simulink model "rfsoc4x2_ospfb_128"  (R2021a)
settings: Solver=VariableStepAuto  StartTime=0.0  StopTime=2048  RelTol=1e-3
undefined symbols (not defined in the file): pfb_coeff_gen_calc
libraries: xbsIndex_r4 x37092, casper_library_delays x737, casper_library_misc x68, xps_library x1
(part 335 of 339)

== system rfsoc4x2_ospfb_128/fft2/fft_biplex/biplex_core/fft_stage_4/butterfly_direct/twiddle/bus_mult/mult4/a_replicate ==
  in : Inport
  bussify : Subsystem  AncestorBlock=casper_library_flow_control/bus_create  mask(bus_create){inputNum=2}
      mask prompts: inputNum "Number of inputs:"
      mask init:
      | bus_create_init(gcb,...
      |     'inputNum', inputNum);
  out : Outport
  wires:
  bussify/1(bus_out) -> out/1
  in/1 -> bussify/2(in2), bussify/1(in1)

== system rfsoc4x2_ospfb_128/fft2/fft_biplex/biplex_core/fft_stage_4/butterfly_direct/twiddle/bus_mult/mult4/b_expand ==
  bus_in : Inport
  reinterpret{1..4} (4 alike) : xbsIndex_r4/Reinterpret  force_arith_type=on  arith_type="Signed  (2's comp)"  force_bin_pt=on  bin_pt=17  block_type=reinterpret
  slice1 : xbsIndex_r4/Slice  nbits=18  boolean_output=off  mode=Upper Bit Location + Width  bit1=-54  base1=MSB of Input  bit0=0  base0=LSB of Input  dbl_ovrd=off  block_type=slice
  slice2 : xbsIndex_r4/Slice  nbits=18  boolean_output=off  mode=Upper Bit Location + Width  bit1=-36  base1=MSB of Input  bit0=0  base0=LSB of Input  dbl_ovrd=off  block_type=slice
  slice3 : xbsIndex_r4/Slice  nbits=18  boolean_output=off  mode=Upper Bit Location + Width  bit1=-18  base1=MSB of Input  bit0=0  base0=LSB of Input  dbl_ovrd=off  block_type=slice
  slice4 : xbsIndex_r4/Slice  nbits=18  boolean_output=off  mode=Upper Bit Location + Width  bit1=0  base1=MSB of Input  bit0=0  base0=LSB of Input  dbl_ovrd=off  block_type=slice
  msb_out4 : Outport
  out3 : Outport  Port=2
  out2 : Outport  Port=3
  lsb_out1 : Outport  Port=4  VectorParamsAs1DForOutWhenUnconnected=off
  wires:
  reinterpret1/1 -> lsb_out1/1
  slice1/1 -> reinterpret1/1
  reinterpret2/1 -> out2/1
  slice2/1 -> reinterpret2/1
  reinterpret3/1 -> out3/1
  slice3/1 -> reinterpret3/1
  reinterpret4/1 -> msb_out4/1
  slice4/1 -> reinterpret4/1
  bus_in/1 -> slice1/1, slice2/1, slice3/1, slice4/1

== system rfsoc4x2_ospfb_128/fft2/fft_biplex/biplex_core/fft_stage_4/butterfly_direct/twiddle/bus_mult/mult4/b_replicate ==
  in : Inport
  bussify : Subsystem  AncestorBlock=casper_library_flow_control/bus_create  mask(bus_create){inputNum=2}
      mask prompts: inputNum "Number of inputs:"
      mask init:
      | bus_create_init(gcb,...
      |     'inputNum', inputNum);
  out : Outport
  wires:
  bussify/1(bus_out) -> out/1
  in/1 -> bussify/2(in2), bussify/1(in1)

== system rfsoc4x2_ospfb_128/fft2/fft_biplex/biplex_core/fft_stage_4/butterfly_direct/twiddle/bus_mult/mult4/ri_to_c ==
  re : Inport
  im : Inport  Port=2
  concat : xbsIndex_r4/Concat  num_inputs=2  dbl_ovrd=off  block_type=concat
      settings: block_version=9.1.01
  force_im : xbsIndex_r4/Reinterpret  force_arith_type=on  arith_type=Unsigned  force_bin_pt=on  bin_pt=0  block_type=reinterpret
      settings: infoedit="Changes signal type without altering the binary representation.   You can changed the signal between signed and unsigned, and relocate the binary point.<P><P>Hardware notes: In hardware this block costs nothing.<P><P>Example:  Suppose the input is 6 bits wide, signed, with 2 fractional bits, and the output is forced to unsigned with 0 fractional bits.  Then an input of -2.0 (1110.00 in binary 2's complement) becomes an output of 56 (111000 in binary)."  block_version=9.1.01
  force_re : xbsIndex_r4/Reinterpret  force_arith_type=on  arith_type=Unsigned  force_bin_pt=on  bin_pt=0  block_type=reinterpret
      settings: infoedit="Changes signal type without altering the binary representation.   You can changed the signal between signed and unsigned, and relocate the binary point.<P><P>Hardware notes: In hardware this block costs nothing.<P><P>Example:  Suppose the input is 6 bits wide, signed, with 2 fractional bits, and the output is forced to unsigned with 0 fractional bits.  Then an input of -2.0 (1110.00 in binary 2's complement) becomes an output of 56 (111000 in binary)."  block_version=9.1.01
  c : Outport  VectorParamsAs1DForOutWhenUnconnected=off
  wires:
  im/1 -> force_im/1
  concat/1 -> c/1
  re/1 -> force_re/1
  force_im/1 -> concat/2
  force_re/1 -> concat/1

== system rfsoc4x2_ospfb_128/fft2/fft_biplex/biplex_core/fft_stage_4/butterfly_direct/twiddle/bus_mult/repa/bussify ==
  in1 : Inport
  reinterpret1 : xbsIndex_r4/Reinterpret  force_arith_type=on  arith_type=Unsigned  force_bin_pt=on  bin_pt=0  block_type=reinterpret
      settings: infoedit="Changes signal type without altering the binary representation.   You can changed the signal between signed and unsigned, and relocate the binary point.<br><br>Hardware notes: In hardware this block costs nothing.<br><br>Example:  Suppose the input is 6 bits wide, signed, with 2 fractional bits, and the output is forced to unsigned with 0 fractional bits.  Then an input of -2.0 (1110.00 in binary 2's complement) becomes an output of 56 (111000 in binary)."
  bus_out : Outport  VectorParamsAs1DForOutWhenUnconnected=off
  wires:
  reinterpret1/1 -> bus_out/1
  in1/1 -> reinterpret1/1

== system rfsoc4x2_ospfb_128/fft2/fft_biplex/biplex_core/fft_stage_4/butterfly_direct/twiddle/bus_mult/repb/bussify ==
  in1 : Inport
  reinterpret1 : xbsIndex_r4/Reinterpret  force_arith_type=on  arith_type=Unsigned  force_bin_pt=on  bin_pt=0  block_type=reinterpret
      settings: infoedit="Changes signal type without altering the binary representation.   You can changed the signal between signed and unsigned, and relocate the binary point.<br><br>Hardware notes: In hardware this block costs nothing.<br><br>Example:  Suppose the input is 6 bits wide, signed, with 2 fractional bits, and the output is forced to unsigned with 0 fractional bits.  Then an input of -2.0 (1110.00 in binary 2's complement) becomes an output of 56 (111000 in binary)."
  bus_out : Outport  VectorParamsAs1DForOutWhenUnconnected=off
  wires:
  reinterpret1/1 -> bus_out/1
  in1/1 -> reinterpret1/1

== system rfsoc4x2_ospfb_128/fft2/fft_biplex/biplex_core/fft_stage_4/butterfly_direct/twiddle/coeff_gen/cosin/add_convert0 ==
  theta : Inport
  misci : Inport  Port=2
  AddSub5 : xbsIndex_r4/AddSub  mode=Addition  use_carryin=off  use_carryout=off  en=off  latency=0  precision=User Defined  arith_type=Unsigned  n_bits=2  bin_pt=0  quantization=Truncate  overflow=Wrap  use_behavioral_HDL=off  hw_selection=Fabric  pipelined=off  dbl_ovrd=off  block_type=addsub
  Concat : xbsIndex_r4/Concat  num_inputs=2  dbl_ovrd=off  block_type=concat
  Convert2 : xbsIndex_r4/Convert  gui_display_data_type=Fixed-point  arith_type=Unsigned  n_bits=3  bin_pt=0  float_type=Single  exp_bits=8  fraction_bits=24  quantization=Truncate  overflow=Saturate  en=off  latency=conv_latency  pipeline=on  dbl_ovrd=off  block_type=convert
  Delay1 : xbsIndex_r4/Delay  rst=off  infoeditControl=Selection of Reset will increase slice count due to use of real FFs and instead of SRLs  en=off  latency=mux_latency+add_latency+conv_latency  reg_retiming=on  dbl_ovrd=off  block_type=delay
  Delay13 : xbsIndex_r4/Delay  rst=off  infoeditControl=Selection of Reset will increase slice count due to use of real FFs and instead of SRLs  en=off  latency=mux_latency  reg_retiming=on  dbl_ovrd=off  block_type=delay
  Delay14 : xbsIndex_r4/Delay  rst=off  infoeditControl=Selection of Reset will increase slice count due to use of real FFs and instead of SRLs  en=off  latency=add_latency  reg_retiming=off  dbl_ovrd=off  block_type=delay
  Delay2 : xbsIndex_r4/Delay  rst=off  infoeditControl=Selection of Reset will increase slice count due to use of real FFs and instead of SRLs  en=off  latency=add_latency+mux_latency+conv_latency  reg_retiming=on  dbl_ovrd=off  block_type=delay
  direction_offset : xbsIndex_r4/Constant  const=0  gui_display_data_type=Fixed-point  arith_type=Unsigned  n_bits=2  bin_pt=0  preci_type=Single  exp_width=8  frac_width=24  explicit_period=off  period=1  equ=P=C  opselect=C  inp2=PCIN>>17  opr=+  inp1=P  carry=CIN  dbl_ovrd=off  block_type=constant
  fluff : xbsIndex_r4/Concat  num_inputs=2  dbl_ovrd=off  block_type=concat
  invert : xbsIndex_r4/Slice  nbits=1  boolean_output=on  mode=Upper Bit Location + Width  bit1=0  base1=MSB of Input  bit0=0  base0=LSB of Input  dbl_ovrd=off  block_type=slice
  lookup : xbsIndex_r4/Slice  nbits=2  boolean_output=off  mode=Lower Bit Location + Width  bit1=0  base1=MSB of Input  bit0=0  base0=LSB of Input  dbl_ovrd=off  block_type=slice
  new_add : xbsIndex_r4/Slice  nbits=3  boolean_output=off  mode=Lower Bit Location + Width  bit1=0  base1=MSB of Input  bit0=0  base0=LSB of Input  dbl_ovrd=off  block_type=slice
  pad : xbsIndex_r4/Constant  const=0  gui_display_data_type=Fixed-point  arith_type=Unsigned  n_bits=1  bin_pt=0  preci_type=Single  exp_width=8  frac_width=24  explicit_period=off  period=1  equ=P=C  opselect=C  inp2=PCIN>>17  opr=+  inp1=P  carry=CIN  dbl_ovrd=off  block_type=constant
  quadrant : xbsIndex_r4/Slice  nbits=2  boolean_output=off  mode=Upper Bit Location + Width  bit1=0  base1=MSB of Input  bit0=0  base0=LSB of Input  dbl_ovrd=off  block_type=slice
  negate : Outport
  add : Outport  Port=2
  misco : Outport  Port=3
  wires:
  theta/1 -> fluff/2
  pad/1 -> fluff/1
  fluff/1 -> quadrant/1, lookup/1
  direction_offset/1 -> AddSub5/1
  quadrant/1 -> AddSub5/2
  lookup/1 -> Concat/2
  AddSub5/1 -> Concat/1, invert/1
  Concat/1 -> new_add/1
  new_add/1 -> Delay14/1
  Convert2/1 -> add/1
  Delay14/1 -> Delay13/1
  Delay13/1 -> Convert2/1
  invert/1 -> Delay2/1
  Delay2/1 -> negate/1
  misci/1 -> Delay1/1
  Delay1/1 -> misco/1

== system rfsoc4x2_ospfb_128/fft2/fft_biplex/biplex_core/fft_stage_4/butterfly_direct/twiddle/coeff_gen/cosin/add_convert1 ==
  theta : Inport
  misci : Inport  Port=2
  AddSub5 : xbsIndex_r4/AddSub  mode=Addition  use_carryin=off  use_carryout=off  en=off  latency=0  precision=User Defined  arith_type=Unsigned  n_bits=2  bin_pt=0  quantization=Truncate  overflow=Wrap  use_behavioral_HDL=off  hw_selection=Fabric  pipelined=off  dbl_ovrd=off  block_type=addsub
  Concat : xbsIndex_r4/Concat  num_inputs=2  dbl_ovrd=off  block_type=concat
  Convert2 : xbsIndex_r4/Convert  gui_display_data_type=Fixed-point  arith_type=Unsigned  n_bits=3  bin_pt=0  float_type=Single  exp_bits=8  fraction_bits=24  quantization=Truncate  overflow=Saturate  en=off  latency=conv_latency  pipeline=on  dbl_ovrd=off  block_type=convert
  Delay1 : xbsIndex_r4/Delay  rst=off  infoeditControl=Selection of Reset will increase slice count due to use of real FFs and instead of SRLs  en=off  latency=mux_latency+add_latency+conv_latency  reg_retiming=on  dbl_ovrd=off  block_type=delay
  Delay13 : xbsIndex_r4/Delay  rst=off  infoeditControl=Selection of Reset will increase slice count due to use of real FFs and instead of SRLs  en=off  latency=mux_latency  reg_retiming=on  dbl_ovrd=off  block_type=delay
  Delay14 : xbsIndex_r4/Delay  rst=off  infoeditControl=Selection of Reset will increase slice count due to use of real FFs and instead of SRLs  en=off  latency=add_latency  reg_retiming=off  dbl_ovrd=off  block_type=delay
  Delay2 : xbsIndex_r4/Delay  rst=off  infoeditControl=Selection of Reset will increase slice count due to use of real FFs and instead of SRLs  en=off  latency=add_latency+mux_latency+conv_latency  reg_retiming=on  dbl_ovrd=off  block_type=delay
  direction_offset : xbsIndex_r4/Constant  const=0  gui_display_data_type=Fixed-point  arith_type=Unsigned  n_bits=2  bin_pt=0  preci_type=Single  exp_width=8  frac_width=24  explicit_period=off  period=1  equ=P=C  opselect=C  inp2=PCIN>>17  opr=+  inp1=P  carry=CIN  dbl_ovrd=off  block_type=constant
  fluff : xbsIndex_r4/Concat  num_inputs=2  dbl_ovrd=off  block_type=concat
  invert : xbsIndex_r4/Slice  nbits=1  boolean_output=on  mode=Upper Bit Location + Width  bit1=0  base1=MSB of Input  bit0=0  base0=LSB of Input  dbl_ovrd=off  block_type=slice
  lookup : xbsIndex_r4/Slice  nbits=2  boolean_output=off  mode=Lower Bit Location + Width  bit1=0  base1=MSB of Input  bit0=0  base0=LSB of Input  dbl_ovrd=off  block_type=slice
  new_add : xbsIndex_r4/Slice  nbits=3  boolean_output=off  mode=Lower Bit Location + Width  bit1=0  base1=MSB of Input  bit0=0  base0=LSB of Input  dbl_ovrd=off  block_type=slice
  pad : xbsIndex_r4/Constant  const=0  gui_display_data_type=Fixed-point  arith_type=Unsigned  n_bits=1  bin_pt=0  preci_type=Single  exp_width=8  frac_width=24  explicit_period=off  period=1  equ=P=C  opselect=C  inp2=PCIN>>17  opr=+  inp1=P  carry=CIN  dbl_ovrd=off  block_type=constant
  quadrant : xbsIndex_r4/Slice  nbits=2  boolean_output=off  mode=Upper Bit Location + Width  bit1=0  base1=MSB of Input  bit0=0  base0=LSB of Input  dbl_ovrd=off  block_type=slice
  negate : Outport
  add : Outport  Port=2
  misco : Outport  Port=3
  wires:
  theta/1 -> fluff/2
  pad/1 -> fluff/1
  fluff/1 -> quadrant/1, lookup/1
  direction_offset/1 -> AddSub5/1
  quadrant/1 -> AddSub5/2
  lookup/1 -> Concat/2
  AddSub5/1 -> Concat/1, invert/1
  Concat/1 -> new_add/1
  new_add/1 -> Delay14/1
  Convert2/1 -> add/1
  Delay14/1 -> Delay13/1
  Delay13/1 -> Convert2/1
  invert/1 -> Delay2/1
  Delay2/1 -> negate/1
  misci/1 -> Delay1/1
  Delay1/1 -> misco/1

== system rfsoc4x2_ospfb_128/fft2/fft_biplex/biplex_core/fft_stage_4/butterfly_direct/twiddle/coeff_gen/cosin/invert0 ==
  negate : Inport
  in : Inport  Port=2
  misci : Inport  Port=3
  Delay1 : xbsIndex_r4/Delay  rst=off  infoeditControl=Selection of Reset will increase slice count due to use of real FFs and instead of SRLs  en=off  latency=mux_latency+neg_latency  reg_retiming=on  dbl_ovrd=off  block_type=delay
  Delay20 : xbsIndex_r4/Delay  rst=off  infoeditControl=Selection of Reset will increase slice count due to use of real FFs and instead of SRLs  en=off  latency=neg_latency  reg_retiming=on  dbl_ovrd=off  block_type=delay
  Delay21 : xbsIndex_r4/Delay  rst=off  infoeditControl=Selection of Reset will increase slice count due to use of real FFs and instead of SRLs  en=off  latency=neg_latency  reg_retiming=on  dbl_ovrd=off  block_type=delay
  Negate : xbsIndex_r4/Negate  precision=User Defined  arith_type="Signed  (2's comp)"  n_bits=n_bits  bin_pt=bin_pt  quantization=Truncate  overflow=Saturate  en=off  latency=neg_latency  dbl_ovrd=off  block_type=negate
  mux : xbsIndex_r4/Mux  inputs=2  en=off  latency=mux_latency  precision=Full  arith_type=Unsigned  n_bits=16  bin_pt=14  quantization=Truncate  overflow=Wrap  dbl_ovrd=off  block_type=mux
  out : Outport
  misco : Outport  Port=2
  wires:
  misci/1 -> Delay1/1
  negate/1 -> Delay21/1
  in/1 -> Negate/1, Delay20/1
  Delay21/1 -> mux/1
  Delay20/1 -> mux/2
  Negate/1 -> mux/3
  mux/1 -> out/1
  Delay1/1 -> misco/1

== system rfsoc4x2_ospfb_128/fft2/fft_biplex/biplex_core/fft_stage_4/butterfly_direct/twiddle/coeff_gen/cosin/invert1 ==
  negate : Inport
  in : Inport  Port=2
  misci : Inport  Port=3
  Delay1 : xbsIndex_r4/Delay  rst=off  infoeditControl=Selection of Reset will increase slice count due to use of real FFs and instead of SRLs  en=off  latency=mux_latency+neg_latency  reg_retiming=on  dbl_ovrd=off  block_type=delay
  Delay20 : xbsIndex_r4/Delay  rst=off  infoeditControl=Selection of Reset will increase slice count due to use of real FFs and instead of SRLs  en=off  latency=neg_latency  reg_retiming=on  dbl_ovrd=off  block_type=delay
  Delay21 : xbsIndex_r4/Delay  rst=off  infoeditControl=Selection of Reset will increase slice count due to use of real FFs and instead of SRLs  en=off  latency=neg_latency  reg_retiming=on  dbl_ovrd=off  block_type=delay
  Negate : xbsIndex_r4/Negate  precision=User Defined  arith_type="Signed  (2's comp)"  n_bits=n_bits  bin_pt=bin_pt  quantization=Truncate  overflow=Saturate  en=off  latency=neg_latency  dbl_ovrd=off  block_type=negate
  mux : xbsIndex_r4/Mux  inputs=2  en=off  latency=mux_latency  precision=Full  arith_type=Unsigned  n_bits=16  bin_pt=14  quantization=Truncate  overflow=Wrap  dbl_ovrd=off  block_type=mux
  out : Outport
  misco : Outport  Port=2
  wires:
  misci/1 -> Delay1/1
  negate/1 -> Delay21/1
  in/1 -> Negate/1, Delay20/1
  Delay21/1 -> mux/1
  Delay20/1 -> mux/2
  Negate/1 -> mux/3
  mux/1 -> out/1
  Delay1/1 -> misco/1

== system rfsoc4x2_ospfb_128/fft2/fft_biplex/biplex_core/fft_stage_5/butterfly_direct/twiddle/bus_mult/mult1/a_expand ==
  bus_in : Inport
  reinterpret{1..4} (4 alike) : xbsIndex_r4/Reinterpret  force_arith_type=on  arith_type="Signed  (2's comp)"  force_bin_pt=on  bin_pt=17  block_type=reinterpret
  slice1 : xbsIndex_r4/Slice  nbits=18  boolean_output=off  mode=Upper Bit Location + Width  bit1=-54  base1=MSB of Input  bit0=0  base0=LSB of Input  dbl_ovrd=off  block_type=slice
  slice2 : xbsIndex_r4/Slice  nbits=18  boolean_output=off  mode=Upper Bit Location + Width  bit1=-36  base1=MSB of Input  bit0=0  base0=LSB of Input  dbl_ovrd=off  block_type=slice
  slice3 : xbsIndex_r4/Slice  nbits=18  boolean_output=off  mode=Upper Bit Location + Width  bit1=-18  base1=MSB of Input  bit0=0  base0=LSB of Input  dbl_ovrd=off  block_type=slice
  slice4 : xbsIndex_r4/Slice  nbits=18  boolean_output=off  mode=Upper Bit Location + Width  bit1=0  base1=MSB of Input  bit0=0  base0=LSB of Input  dbl_ovrd=off  block_type=slice
  msb_out4 : Outport
  out3 : Outport  Port=2
  out2 : Outport  Port=3
  lsb_out1 : Outport  Port=4  VectorParamsAs1DForOutWhenUnconnected=off
  wires:
  reinterpret1/1 -> lsb_out1/1
  slice1/1 -> reinterpret1/1
  reinterpret2/1 -> out2/1
  slice2/1 -> reinterpret2/1
  reinterpret3/1 -> out3/1
  slice3/1 -> reinterpret3/1
  reinterpret4/1 -> msb_out4/1
  slice4/1 -> reinterpret4/1
  bus_in/1 -> slice1/1, slice2/1, slice3/1, slice4/1

== system rfsoc4x2_ospfb_128/fft2/fft_biplex/biplex_core/fft_stage_5/butterfly_direct/twiddle/bus_mult/mult1/a_replicate ==
  in : Inport
  bussify : Subsystem  AncestorBlock=casper_library_flow_control/bus_create  mask(bus_create){inputNum=2}
      mask prompts: inputNum "Number of inputs:"
      mask init:
      | bus_create_init(gcb,...
      |     'inputNum', inputNum);
  out : Outport
  wires:
  bussify/1(bus_out) -> out/1
  in/1 -> bussify/2(in2), bussify/1(in1)

== system rfsoc4x2_ospfb_128/fft2/fft_biplex/biplex_core/fft_stage_5/butterfly_direct/twiddle/bus_mult/mult1/b_expand ==
  bus_in : Inport
  reinterpret{1..4} (4 alike) : xbsIndex_r4/Reinterpret  force_arith_type=on  arith_type="Signed  (2's comp)"  force_bin_pt=on  bin_pt=17  block_type=reinterpret
  slice1 : xbsIndex_r4/Slice  nbits=18  boolean_output=off  mode=Upper Bit Location + Width  bit1=-54  base1=MSB of Input  bit0=0  base0=LSB of Input  dbl_ovrd=off  block_type=slice
  slice2 : xbsIndex_r4/Slice  nbits=18  boolean_output=off  mode=Upper Bit Location + Width  bit1=-36  base1=MSB of Input  bit0=0  base0=LSB of Input  dbl_ovrd=off  block_type=slice
  slice3 : xbsIndex_r4/Slice  nbits=18  boolean_output=off  mode=Upper Bit Location + Width  bit1=-18  base1=MSB of Input  bit0=0  base0=LSB of Input  dbl_ovrd=off  block_type=slice
  slice4 : xbsIndex_r4/Slice  nbits=18  boolean_output=off  mode=Upper Bit Location + Width  bit1=0  base1=MSB of Input  bit0=0  base0=LSB of Input  dbl_ovrd=off  block_type=slice
  msb_out4 : Outport
  out3 : Outport  Port=2
  out2 : Outport  Port=3
  lsb_out1 : Outport  Port=4  VectorParamsAs1DForOutWhenUnconnected=off
  wires:
  reinterpret1/1 -> lsb_out1/1
  slice1/1 -> reinterpret1/1
  reinterpret2/1 -> out2/1
  slice2/1 -> reinterpret2/1
  reinterpret3/1 -> out3/1
  slice3/1 -> reinterpret3/1
  reinterpret4/1 -> msb_out4/1
  slice4/1 -> reinterpret4/1
  bus_in/1 -> slice1/1, slice2/1, slice3/1, slice4/1

== system rfsoc4x2_ospfb_128/fft2/fft_biplex/biplex_core/fft_stage_5/butterfly_direct/twiddle/bus_mult/mult1/b_replicate ==
  in : Inport
  bussify : Subsystem  AncestorBlock=casper_library_flow_control/bus_create  mask(bus_create){inputNum=2}
      mask prompts: inputNum "Number of inputs:"
      mask init:
      | bus_create_init(gcb,...
      |     'inputNum', inputNum);
  out : Outport
  wires:
  bussify/1(bus_out) -> out/1
  in/1 -> bussify/2(in2), bussify/1(in1)

== system rfsoc4x2_ospfb_128/fft2/fft_biplex/biplex_core/fft_stage_5/butterfly_direct/twiddle/bus_mult/mult1/ri_to_c ==
  re : Inport
  im : Inport  Port=2
  concat : xbsIndex_r4/Concat  num_inputs=2  dbl_ovrd=off  block_type=concat
      settings: block_version=9.1.01
  force_im : xbsIndex_r4/Reinterpret  force_arith_type=on  arith_type=Unsigned  force_bin_pt=on  bin_pt=0  block_type=reinterpret
      settings: infoedit="Changes signal type without altering the binary representation.   You can changed the signal between signed and unsigned, and relocate the binary point.<P><P>Hardware notes: In hardware this block costs nothing.<P><P>Example:  Suppose the input is 6 bits wide, signed, with 2 fractional bits, and the output is forced to unsigned with 0 fractional bits.  Then an input of -2.0 (1110.00 in binary 2's complement) becomes an output of 56 (111000 in binary)."  block_version=9.1.01
  force_re : xbsIndex_r4/Reinterpret  force_arith_type=on  arith_type=Unsigned  force_bin_pt=on  bin_pt=0  block_type=reinterpret
      settings: infoedit="Changes signal type without altering the binary representation.   You can changed the signal between signed and unsigned, and relocate the binary point.<P><P>Hardware notes: In hardware this block costs nothing.<P><P>Example:  Suppose the input is 6 bits wide, signed, with 2 fractional bits, and the output is forced to unsigned with 0 fractional bits.  Then an input of -2.0 (1110.00 in binary 2's complement) becomes an output of 56 (111000 in binary)."  block_version=9.1.01
  c : Outport  VectorParamsAs1DForOutWhenUnconnected=off
  wires:
  im/1 -> force_im/1
  concat/1 -> c/1
  re/1 -> force_re/1
  force_im/1 -> concat/2
  force_re/1 -> concat/1

== system rfsoc4x2_ospfb_128/fft2/fft_biplex/biplex_core/fft_stage_5/butterfly_direct/twiddle/bus_mult/mult2/a_expand ==
  bus_in : Inport
  reinterpret{1..4} (4 alike) : xbsIndex_r4/Reinterpret  force_arith_type=on  arith_type="Signed  (2's comp)"  force_bin_pt=on  bin_pt=17  block_type=reinterpret
  slice1 : xbsIndex_r4/Slice  nbits=18  boolean_output=off  mode=Upper Bit Location + Width  bit1=-54  base1=MSB of Input  bit0=0  base0=LSB of Input  dbl_ovrd=off  block_type=slice
  slice2 : xbsIndex_r4/Slice  nbits=18  boolean_output=off  mode=Upper Bit Location + Width  bit1=-36  base1=MSB of Input  bit0=0  base0=LSB of Input  dbl_ovrd=off  block_type=slice
  slice3 : xbsIndex_r4/Slice  nbits=18  boolean_output=off  mode=Upper Bit Location + Width  bit1=-18  base1=MSB of Input  bit0=0  base0=LSB of Input  dbl_ovrd=off  block_type=slice
  slice4 : xbsIndex_r4/Slice  nbits=18  boolean_output=off  mode=Upper Bit Location + Width  bit1=0  base1=MSB of Input  bit0=0  base0=LSB of Input  dbl_ovrd=off  block_type=slice
  msb_out4 : Outport
  out3 : Outport  Port=2
  out2 : Outport  Port=3
  lsb_out1 : Outport  Port=4  VectorParamsAs1DForOutWhenUnconnected=off
  wires:
  reinterpret1/1 -> lsb_out1/1
  slice1/1 -> reinterpret1/1
  reinterpret2/1 -> out2/1
  slice2/1 -> reinterpret2/1
  reinterpret3/1 -> out3/1
  slice3/1 -> reinterpret3/1
  reinterpret4/1 -> msb_out4/1
  slice4/1 -> reinterpret4/1
  bus_in/1 -> slice1/1, slice2/1, slice3/1, slice4/1

== system rfsoc4x2_ospfb_128/fft2/fft_biplex/biplex_core/fft_stage_5/butterfly_direct/twiddle/bus_mult/mult2/a_replicate ==
  in : Inport
  bussify : Subsystem  AncestorBlock=casper_library_flow_control/bus_create  mask(bus_create){inputNum=2}
      mask prompts: inputNum "Number of inputs:"
      mask init:
      | bus_create_init(gcb,...
      |     'inputNum', inputNum);
  out : Outport
  wires:
  bussify/1(bus_out) -> out/1
  in/1 -> bussify/2(in2), bussify/1(in1)

== system rfsoc4x2_ospfb_128/fft2/fft_biplex/biplex_core/fft_stage_5/butterfly_direct/twiddle/bus_mult/mult2/b_expand ==
  bus_in : Inport
  reinterpret{1..4} (4 alike) : xbsIndex_r4/Reinterpret  force_arith_type=on  arith_type="Signed  (2's comp)"  force_bin_pt=on  bin_pt=17  block_type=reinterpret
  slice1 : xbsIndex_r4/Slice  nbits=18  boolean_output=off  mode=Upper Bit Location + Width  bit1=-54  base1=MSB of Input  bit0=0  base0=LSB of Input  dbl_ovrd=off  block_type=slice
  slice2 : xbsIndex_r4/Slice  nbits=18  boolean_output=off  mode=Upper Bit Location + Width  bit1=-36  base1=MSB of Input  bit0=0  base0=LSB of Input  dbl_ovrd=off  block_type=slice
  slice3 : xbsIndex_r4/Slice  nbits=18  boolean_output=off  mode=Upper Bit Location + Width  bit1=-18  base1=MSB of Input  bit0=0  base0=LSB of Input  dbl_ovrd=off  block_type=slice
  slice4 : xbsIndex_r4/Slice  nbits=18  boolean_output=off  mode=Upper Bit Location + Width  bit1=0  base1=MSB of Input  bit0=0  base0=LSB of Input  dbl_ovrd=off  block_type=slice
  msb_out4 : Outport
  out3 : Outport  Port=2
  out2 : Outport  Port=3
  lsb_out1 : Outport  Port=4  VectorParamsAs1DForOutWhenUnconnected=off
  wires:
  reinterpret1/1 -> lsb_out1/1
  slice1/1 -> reinterpret1/1
  reinterpret2/1 -> out2/1
  slice2/1 -> reinterpret2/1
  reinterpret3/1 -> out3/1
  slice3/1 -> reinterpret3/1
  reinterpret4/1 -> msb_out4/1
  slice4/1 -> reinterpret4/1
  bus_in/1 -> slice1/1, slice2/1, slice3/1, slice4/1

== system rfsoc4x2_ospfb_128/fft2/fft_biplex/biplex_core/fft_stage_5/butterfly_direct/twiddle/bus_mult/mult2/b_replicate ==
  in : Inport
  bussify : Subsystem  AncestorBlock=casper_library_flow_control/bus_create  mask(bus_create){inputNum=2}
      mask prompts: inputNum "Number of inputs:"
      mask init:
      | bus_create_init(gcb,...
      |     'inputNum', inputNum);
  out : Outport
  wires:
  bussify/1(bus_out) -> out/1
  in/1 -> bussify/2(in2), bussify/1(in1)

== system rfsoc4x2_ospfb_128/fft2/fft_biplex/biplex_core/fft_stage_5/butterfly_direct/twiddle/bus_mult/mult2/ri_to_c ==
  re : Inport
  im : Inport  Port=2
  concat : xbsIndex_r4/Concat  num_inputs=2  dbl_ovrd=off  block_type=concat
      settings: block_version=9.1.01
  force_im : xbsIndex_r4/Reinterpret  force_arith_type=on  arith_type=Unsigned  force_bin_pt=on  bin_pt=0  block_type=reinterpret
      settings: infoedit="Changes signal type without altering the binary representation.   You can changed the signal between signed and unsigned, and relocate the binary point.<P><P>Hardware notes: In hardware this block costs nothing.<P><P>Example:  Suppose the input is 6 bits wide, signed, with 2 fractional bits, and the output is forced to unsigned with 0 fractional bits.  Then an input of -2.0 (1110.00 in binary 2's complement) becomes an output of 56 (111000 in binary)."  block_version=9.1.01
  force_re : xbsIndex_r4/Reinterpret  force_arith_type=on  arith_type=Unsigned  force_bin_pt=on  bin_pt=0  block_type=reinterpret
      settings: infoedit="Changes signal type without altering the binary representation.   You can changed the signal between signed and unsigned, and relocate the binary point.<P><P>Hardware notes: In hardware this block costs nothing.<P><P>Example:  Suppose the input is 6 bits wide, signed, with 2 fractional bits, and the output is forced to unsigned with 0 fractional bits.  Then an input of -2.0 (1110.00 in binary 2's complement) becomes an output of 56 (111000 in binary)."  block_version=9.1.01
  c : Outport  VectorParamsAs1DForOutWhenUnconnected=off
  wires:
  im/1 -> force_im/1
  concat/1 -> c/1
  re/1 -> force_re/1
  force_im/1 -> concat/2
  force_re/1 -> concat/1

== system rfsoc4x2_ospfb_128/fft2/fft_biplex/biplex_core/fft_stage_5/butterfly_direct/twiddle/bus_mult/mult3/a_expand ==
  bus_in : Inport
  reinterpret{1..4} (4 alike) : xbsIndex_r4/Reinterpret  force_arith_type=on  arith_type="Signed  (2's comp)"  force_bin_pt=on  bin_pt=17  block_type=reinterpret
  slice1 : xbsIndex_r4/Slice  nbits=18  boolean_output=off  mode=Upper Bit Location + Width  bit1=-54  base1=MSB of Input  bit0=0  base0=LSB of Input  dbl_ovrd=off  block_type=slice
  slice2 : xbsIndex_r4/Slice  nbits=18  boolean_output=off  mode=Upper Bit Location + Width  bit1=-36  base1=MSB of Input  bit0=0  base0=LSB of Input  dbl_ovrd=off  block_type=slice
  slice3 : xbsIndex_r4/Slice  nbits=18  boolean_output=off  mode=Upper Bit Location + Width  bit1=-18  base1=MSB of Input  bit0=0  base0=LSB of Input  dbl_ovrd=off  block_type=slice
  slice4 : xbsIndex_r4/Slice  nbits=18  boolean_output=off  mode=Upper Bit Location + Width  bit1=0  base1=MSB of Input  bit0=0  base0=LSB of Input  dbl_ovrd=off  block_type=slice
  msb_out4 : Outport
  out3 : Outport  Port=2
  out2 : Outport  Port=3
  lsb_out1 : Outport  Port=4  VectorParamsAs1DForOutWhenUnconnected=off
  wires:
  reinterpret1/1 -> lsb_out1/1
  slice1/1 -> reinterpret1/1
  reinterpret2/1 -> out2/1
  slice2/1 -> reinterpret2/1
  reinterpret3/1 -> out3/1
  slice3/1 -> reinterpret3/1
  reinterpret4/1 -> msb_out4/1
  slice4/1 -> reinterpret4/1
  bus_in/1 -> slice1/1, slice2/1, slice3/1, slice4/1

== system rfsoc4x2_ospfb_128/fft2/fft_biplex/biplex_core/fft_stage_5/butterfly_direct/twiddle/bus_mult/mult3/a_replicate ==
  in : Inport
  bussify : Subsystem  AncestorBlock=casper_library_flow_control/bus_create  mask(bus_create){inputNum=2}
      mask prompts: inputNum "Number of inputs:"
      mask init:
      | bus_create_init(gcb,...
      |     'inputNum', inputNum);
  out : Outport
  wires:
  bussify/1(bus_out) -> out/1
  in/1 -> bussify/2(in2), bussify/1(in1)

== system rfsoc4x2_ospfb_128/fft2/fft_biplex/biplex_core/fft_stage_5/butterfly_direct/twiddle/bus_mult/mult3/b_expand ==
  bus_in : Inport
  reinterpret{1..4} (4 alike) : xbsIndex_r4/Reinterpret  force_arith_type=on  arith_type="Signed  (2's comp)"  force_bin_pt=on  bin_pt=17  block_type=reinterpret
  slice1 : xbsIndex_r4/Slice  nbits=18  boolean_output=off  mode=Upper Bit Location + Width  bit1=-54  base1=MSB of Input  bit0=0  base0=LSB of Input  dbl_ovrd=off  block_type=slice
  slice2 : xbsIndex_r4/Slice  nbits=18  boolean_output=off  mode=Upper Bit Location + Width  bit1=-36  base1=MSB of Input  bit0=0  base0=LSB of Input  dbl_ovrd=off  block_type=slice
  slice3 : xbsIndex_r4/Slice  nbits=18  boolean_output=off  mode=Upper Bit Location + Width  bit1=-18  base1=MSB of Input  bit0=0  base0=LSB of Input  dbl_ovrd=off  block_type=slice
  slice4 : xbsIndex_r4/Slice  nbits=18  boolean_output=off  mode=Upper Bit Location + Width  bit1=0  base1=MSB of Input  bit0=0  base0=LSB of Input  dbl_ovrd=off  block_type=slice
  msb_out4 : Outport
  out3 : Outport  Port=2
  out2 : Outport  Port=3
  lsb_out1 : Outport  Port=4  VectorParamsAs1DForOutWhenUnconnected=off
  wires:
  reinterpret1/1 -> lsb_out1/1
  slice1/1 -> reinterpret1/1
  reinterpret2/1 -> out2/1
  slice2/1 -> reinterpret2/1
  reinterpret3/1 -> out3/1
  slice3/1 -> reinterpret3/1
  reinterpret4/1 -> msb_out4/1
  slice4/1 -> reinterpret4/1
  bus_in/1 -> slice1/1, slice2/1, slice3/1, slice4/1

== system rfsoc4x2_ospfb_128/fft2/fft_biplex/biplex_core/fft_stage_5/butterfly_direct/twiddle/bus_mult/mult3/b_replicate ==
  in : Inport
  bussify : Subsystem  AncestorBlock=casper_library_flow_control/bus_create  mask(bus_create){inputNum=2}
      mask prompts: inputNum "Number of inputs:"
      mask init:
      | bus_create_init(gcb,...
      |     'inputNum', inputNum);
  out : Outport
  wires:
  bussify/1(bus_out) -> out/1
  in/1 -> bussify/2(in2), bussify/1(in1)

== system rfsoc4x2_ospfb_128/fft2/fft_biplex/biplex_core/fft_stage_5/butterfly_direct/twiddle/bus_mult/mult3/ri_to_c ==
  re : Inport
  im : Inport  Port=2
  concat : xbsIndex_r4/Concat  num_inputs=2  dbl_ovrd=off  block_type=concat
      settings: block_version=9.1.01
  force_im : xbsIndex_r4/Reinterpret  force_arith_type=on  arith_type=Unsigned  force_bin_pt=on  bin_pt=0  block_type=reinterpret
      settings: infoedit="Changes signal type without altering the binary representation.   You can changed the signal between signed and unsigned, and relocate the binary point.<P><P>Hardware notes: In hardware this block costs nothing.<P><P>Example:  Suppose the input is 6 bits wide, signed, with 2 fractional bits, and the output is forced to unsigned with 0 fractional bits.  Then an input of -2.0 (1110.00 in binary 2's complement) becomes an output of 56 (111000 in binary)."  block_version=9.1.01
  force_re : xbsIndex_r4/Reinterpret  force_arith_type=on  arith_type=Unsigned  force_bin_pt=on  bin_pt=0  block_type=reinterpret
      settings: infoedit="Changes signal type without altering the binary representation.   You can changed the signal between signed and unsigned, and relocate the binary point.<P><P>Hardware notes: In hardware this block costs nothing.<P><P>Example:  Suppose the input is 6 bits wide, signed, with 2 fractional bits, and the output is forced to unsigned with 0 fractional bits.  Then an input of -2.0 (1110.00 in binary 2's complement) becomes an output of 56 (111000 in binary)."  block_version=9.1.01
  c : Outport  VectorParamsAs1DForOutWhenUnconnected=off
  wires:
  im/1 -> force_im/1
  concat/1 -> c/1
  re/1 -> force_re/1
  force_im/1 -> concat/2
  force_re/1 -> concat/1

== system rfsoc4x2_ospfb_128/fft2/fft_biplex/biplex_core/fft_stage_5/butterfly_direct/twiddle/bus_mult/mult4/a_expand ==
  bus_in : Inport
  reinterpret{1..4} (4 alike) : xbsIndex_r4/Reinterpret  force_arith_type=on  arith_type="Signed  (2's comp)"  force_bin_pt=on  bin_pt=17  block_type=reinterpret
  slice1 : xbsIndex_r4/Slice  nbits=18  boolean_output=off  mode=Upper Bit Location + Width  bit1=-54  base1=MSB of Input  bit0=0  base0=LSB of Input  dbl_ovrd=off  block_type=slice
  slice2 : xbsIndex_r4/Slice  nbits=18  boolean_output=off  mode=Upper Bit Location + Width  bit1=-36  base1=MSB of Input  bit0=0  base0=LSB of Input  dbl_ovrd=off  block_type=slice
  slice3 : xbsIndex_r4/Slice  nbits=18  boolean_output=off  mode=Upper Bit Location + Width  bit1=-18  base1=MSB of Input  bit0=0  base0=LSB of Input  dbl_ovrd=off  block_type=slice
  slice4 : xbsIndex_r4/Slice  nbits=18  boolean_output=off  mode=Upper Bit Location + Width  bit1=0  base1=MSB of Input  bit0=0  base0=LSB of Input  dbl_ovrd=off  block_type=slice
  msb_out4 : Outport
  out3 : Outport  Port=2
  out2 : Outport  Port=3
  lsb_out1 : Outport  Port=4  VectorParamsAs1DForOutWhenUnconnected=off
  wires:
  reinterpret1/1 -> lsb_out1/1
  slice1/1 -> reinterpret1/1
  reinterpret2/1 -> out2/1
  slice2/1 -> reinterpret2/1
  reinterpret3/1 -> out3/1
  slice3/1 -> reinterpret3/1
  reinterpret4/1 -> msb_out4/1
  slice4/1 -> reinterpret4/1
  bus_in/1 -> slice1/1, slice2/1, slice3/1, slice4/1

== system rfsoc4x2_ospfb_128/fft2/fft_biplex/biplex_core/fft_stage_5/butterfly_direct/twiddle/bus_mult/mult4/a_replicate ==
  in : Inport
  bussify : Subsystem  AncestorBlock=casper_library_flow_control/bus_create  mask(bus_create){inputNum=2}
      mask prompts: inputNum "Number of inputs:"
      mask init:
      | bus_create_init(gcb,...
      |     'inputNum', inputNum);
  out : Outport
  wires:
  bussify/1(bus_out) -> out/1
  in/1 -> bussify/2(in2), bussify/1(in1)

== system rfsoc4x2_ospfb_128/fft2/fft_biplex/biplex_core/fft_stage_5/butterfly_direct/twiddle/bus_mult/mult4/b_expand ==
  bus_in : Inport
  reinterpret{1..4} (4 alike) : xbsIndex_r4/Reinterpret  force_arith_type=on  arith_type="Signed  (2's comp)"  force_bin_pt=on  bin_pt=17  block_type=reinterpret
  slice1 : xbsIndex_r4/Slice  nbits=18  boolean_output=off  mode=Upper Bit Location + Width  bit1=-54  base1=MSB of Input  bit0=0  base0=LSB of Input  dbl_ovrd=off  block_type=slice
  slice2 : xbsIndex_r4/Slice  nbits=18  boolean_output=off  mode=Upper Bit Location + Width  bit1=-36  base1=MSB of Input  bit0=0  base0=LSB of Input  dbl_ovrd=off  block_type=slice
  slice3 : xbsIndex_r4/Slice  nbits=18  boolean_output=off  mode=Upper Bit Location + Width  bit1=-18  base1=MSB of Input  bit0=0  base0=LSB of Input  dbl_ovrd=off  block_type=slice
  slice4 : xbsIndex_r4/Slice  nbits=18  boolean_output=off  mode=Upper Bit Location + Width  bit1=0  base1=MSB of Input  bit0=0  base0=LSB of Input  dbl_ovrd=off  block_type=slice
  msb_out4 : Outport
  out3 : Outport  Port=2
  out2 : Outport  Port=3
  lsb_out1 : Outport  Port=4  VectorParamsAs1DForOutWhenUnconnected=off
  wires:
  reinterpret1/1 -> lsb_out1/1
  slice1/1 -> reinterpret1/1
  reinterpret2/1 -> out2/1
  slice2/1 -> reinterpret2/1
  reinterpret3/1 -> out3/1
  slice3/1 -> reinterpret3/1
  reinterpret4/1 -> msb_out4/1
  slice4/1 -> reinterpret4/1
  bus_in/1 -> slice1/1, slice2/1, slice3/1, slice4/1

== system rfsoc4x2_ospfb_128/fft2/fft_biplex/biplex_core/fft_stage_5/butterfly_direct/twiddle/bus_mult/mult4/b_replicate ==
  in : Inport
  bussify : Subsystem  AncestorBlock=casper_library_flow_control/bus_create  mask(bus_create){inputNum=2}
      mask prompts: inputNum "Number of inputs:"
      mask init:
      | bus_create_init(gcb,...
      |     'inputNum', inputNum);
  out : Outport
  wires:
  bussify/1(bus_out) -> out/1
  in/1 -> bussify/2(in2), bussify/1(in1)

== system rfsoc4x2_ospfb_128/fft2/fft_biplex/biplex_core/fft_stage_5/butterfly_direct/twiddle/bus_mult/mult4/ri_to_c ==
  re : Inport
  im : Inport  Port=2
  concat : xbsIndex_r4/Concat  num_inputs=2  dbl_ovrd=off  block_type=concat
      settings: block_version=9.1.01
  force_im : xbsIndex_r4/Reinterpret  force_arith_type=on  arith_type=Unsigned  force_bin_pt=on  bin_pt=0  block_type=reinterpret
      settings: infoedit="Changes signal type without altering the binary representation.   You can changed the signal between signed and unsigned, and relocate the binary point.<P><P>Hardware notes: In hardware this block costs nothing.<P><P>Example:  Suppose the input is 6 bits wide, signed, with 2 fractional bits, and the output is forced to unsigned with 0 fractional bits.  Then an input of -2.0 (1110.00 in binary 2's complement) becomes an output of 56 (111000 in binary)."  block_version=9.1.01
  force_re : xbsIndex_r4/Reinterpret  force_arith_type=on  arith_type=Unsigned  force_bin_pt=on  bin_pt=0  block_type=reinterpret
      settings: infoedit="Changes signal type without altering the binary representation.   You can changed the signal between signed and unsigned, and relocate the binary point.<P><P>Hardware notes: In hardware this block costs nothing.<P><P>Example:  Suppose the input is 6 bits wide, signed, with 2 fractional bits, and the output is forced to unsigned with 0 fractional bits.  Then an input of -2.0 (1110.00 in binary 2's complement) becomes an output of 56 (111000 in binary)."  block_version=9.1.01
  c : Outport  VectorParamsAs1DForOutWhenUnconnected=off
  wires:
  im/1 -> force_im/1
  concat/1 -> c/1
  re/1 -> force_re/1
  force_im/1 -> concat/2
  force_re/1 -> concat/1

== system rfsoc4x2_ospfb_128/fft2/fft_biplex/biplex_core/fft_stage_5/butterfly_direct/twiddle/bus_mult/repa/bussify ==
  in1 : Inport
  reinterpret1 : xbsIndex_r4/Reinterpret  force_arith_type=on  arith_type=Unsigned  force_bin_pt=on  bin_pt=0  block_type=reinterpret
      settings: infoedit="Changes signal type without altering the binary representation.   You can changed the signal between signed and unsigned, and relocate the binary point.<br><br>Hardware notes: In hardware this block costs nothing.<br><br>Example:  Suppose the input is 6 bits wide, signed, with 2 fractional bits, and the output is forced to unsigned with 0 fractional bits.  Then an input of -2.0 (1110.00 in binary 2's complement) becomes an output of 56 (111000 in binary)."
  bus_out : Outport  VectorParamsAs1DForOutWhenUnconnected=off
  wires:
  reinterpret1/1 -> bus_out/1
  in1/1 -> reinterpret1/1

== system rfsoc4x2_ospfb_128/fft2/fft_biplex/biplex_core/fft_stage_5/butterfly_direct/twiddle/bus_mult/repb/bussify ==
  in1 : Inport
  reinterpret1 : xbsIndex_r4/Reinterpret  force_arith_type=on  arith_type=Unsigned  force_bin_pt=on  bin_pt=0  block_type=reinterpret
      settings: infoedit="Changes signal type without altering the binary representation.   You can changed the signal between signed and unsigned, and relocate the binary point.<br><br>Hardware notes: In hardware this block costs nothing.<br><br>Example:  Suppose the input is 6 bits wide, signed, with 2 fractional bits, and the output is forced to unsigned with 0 fractional bits.  Then an input of -2.0 (1110.00 in binary 2's complement) becomes an output of 56 (111000 in binary)."
  bus_out : Outport  VectorParamsAs1DForOutWhenUnconnected=off
  wires:
  reinterpret1/1 -> bus_out/1
  in1/1 -> reinterpret1/1

== system rfsoc4x2_ospfb_128/fft2/fft_biplex/biplex_core/fft_stage_5/butterfly_direct/twiddle/coeff_gen/cosin/add_convert0 ==
  theta : Inport
  misci : Inport  Port=2
  AddSub5 : xbsIndex_r4/AddSub  mode=Addition  use_carryin=off  use_carryout=off  en=off  latency=0  precision=User Defined  arith_type=Unsigned  n_bits=2  bin_pt=0  quantization=Truncate  overflow=Wrap  use_behavioral_HDL=off  hw_selection=Fabric  pipelined=off  dbl_ovrd=off  block_type=addsub
  Concat : xbsIndex_r4/Concat  num_inputs=2  dbl_ovrd=off  block_type=concat
  Convert2 : xbsIndex_r4/Convert  gui_display_data_type=Fixed-point  arith_type=Unsigned  n_bits=4  bin_pt=0  float_type=Single  exp_bits=8  fraction_bits=24  quantization=Truncate  overflow=Saturate  en=off  latency=conv_latency  pipeline=on  dbl_ovrd=off  block_type=convert
  Delay1 : xbsIndex_r4/Delay  rst=off  infoeditControl=Selection of Reset will increase slice count due to use of real FFs and instead of SRLs  en=off  latency=mux_latency+add_latency+conv_latency  reg_retiming=on  dbl_ovrd=off  block_type=delay
  Delay13 : xbsIndex_r4/Delay  rst=off  infoeditControl=Selection of Reset will increase slice count due to use of real FFs and instead of SRLs  en=off  latency=mux_latency  reg_retiming=on  dbl_ovrd=off  block_type=delay
  Delay14 : xbsIndex_r4/Delay  rst=off  infoeditControl=Selection of Reset will increase slice count due to use of real FFs and instead of SRLs  en=off  latency=add_latency  reg_retiming=off  dbl_ovrd=off  block_type=delay
  Delay2 : xbsIndex_r4/Delay  rst=off  infoeditControl=Selection of Reset will increase slice count due to use of real FFs and instead of SRLs  en=off  latency=add_latency+mux_latency+conv_latency  reg_retiming=on  dbl_ovrd=off  block_type=delay
  direction_offset : xbsIndex_r4/Constant  const=0  gui_display_data_type=Fixed-point  arith_type=Unsigned  n_bits=2  bin_pt=0  preci_type=Single  exp_width=8  frac_width=24  explicit_period=off  period=1  equ=P=C  opselect=C  inp2=PCIN>>17  opr=+  inp1=P  carry=CIN  dbl_ovrd=off  block_type=constant
  fluff : xbsIndex_r4/Concat  num_inputs=2  dbl_ovrd=off  block_type=concat
  invert : xbsIndex_r4/Slice  nbits=1  boolean_output=on  mode=Upper Bit Location + Width  bit1=0  base1=MSB of Input  bit0=0  base0=LSB of Input  dbl_ovrd=off  block_type=slice
  lookup : xbsIndex_r4/Slice  nbits=3  boolean_output=off  mode=Lower Bit Location + Width  bit1=0  base1=MSB of Input  bit0=0  base0=LSB of Input  dbl_ovrd=off  block_type=slice
  new_add : xbsIndex_r4/Slice  nbits=4  boolean_output=off  mode=Lower Bit Location + Width  bit1=0  base1=MSB of Input  bit0=0  base0=LSB of Input  dbl_ovrd=off  block_type=slice
  pad : xbsIndex_r4/Constant  const=0  gui_display_data_type=Fixed-point  arith_type=Unsigned  n_bits=1  bin_pt=0  preci_type=Single  exp_width=8  frac_width=24  explicit_period=off  period=1  equ=P=C  opselect=C  inp2=PCIN>>17  opr=+  inp1=P  carry=CIN  dbl_ovrd=off  block_type=constant
  quadrant : xbsIndex_r4/Slice  nbits=2  boolean_output=off  mode=Upper Bit Location + Width  bit1=0  base1=MSB of Input  bit0=0  base0=LSB of Input  dbl_ovrd=off  block_type=slice
  negate : Outport
  add : Outport  Port=2
  misco : Outport  Port=3
  wires:
  theta/1 -> fluff/2
  pad/1 -> fluff/1
  fluff/1 -> quadrant/1, lookup/1
  direction_offset/1 -> AddSub5/1
  quadrant/1 -> AddSub5/2
  lookup/1 -> Concat/2
  AddSub5/1 -> Concat/1, invert/1
  Concat/1 -> new_add/1
  new_add/1 -> Delay14/1
  Convert2/1 -> add/1
  Delay14/1 -> Delay13/1
  Delay13/1 -> Convert2/1
  invert/1 -> Delay2/1
  Delay2/1 -> negate/1
  misci/1 -> Delay1/1
  Delay1/1 -> misco/1

== system rfsoc4x2_ospfb_128/fft2/fft_biplex/biplex_core/fft_stage_5/butterfly_direct/twiddle/coeff_gen/cosin/add_convert1 ==
  theta : Inport
  misci : Inport  Port=2
  AddSub5 : xbsIndex_r4/AddSub  mode=Addition  use_carryin=off  use_carryout=off  en=off  latency=0  precision=User Defined  arith_type=Unsigned  n_bits=2  bin_pt=0  quantization=Truncate  overflow=Wrap  use_behavioral_HDL=off  hw_selection=Fabric  pipelined=off  dbl_ovrd=off  block_type=addsub
  Concat : xbsIndex_r4/Concat  num_inputs=2  dbl_ovrd=off  block_type=concat
  Convert2 : xbsIndex_r4/Convert  gui_display_data_type=Fixed-point  arith_type=Unsigned  n_bits=4  bin_pt=0  float_type=Single  exp_bits=8  fraction_bits=24  quantization=Truncate  overflow=Saturate  en=off  latency=conv_latency  pipeline=on  dbl_ovrd=off  block_type=convert
  Delay1 : xbsIndex_r4/Delay  rst=off  infoeditControl=Selection of Reset will increase slice count due to use of real FFs and instead of SRLs  en=off  latency=mux_latency+add_latency+conv_latency  reg_retiming=on  dbl_ovrd=off  block_type=delay
  Delay13 : xbsIndex_r4/Delay  rst=off  infoeditControl=Selection of Reset will increase slice count due to use of real FFs and instead of SRLs  en=off  latency=mux_latency  reg_retiming=on  dbl_ovrd=off  block_type=delay
  Delay14 : xbsIndex_r4/Delay  rst=off  infoeditControl=Selection of Reset will increase slice count due to use of real FFs and instead of SRLs  en=off  latency=add_latency  reg_retiming=off  dbl_ovrd=off  block_type=delay
  Delay2 : xbsIndex_r4/Delay  rst=off  infoeditControl=Selection of Reset will increase slice count due to use of real FFs and instead of SRLs  en=off  latency=add_latency+mux_latency+conv_latency  reg_retiming=on  dbl_ovrd=off  block_type=delay
  direction_offset : xbsIndex_r4/Constant  const=0  gui_display_data_type=Fixed-point  arith_type=Unsigned  n_bits=2  bin_pt=0  preci_type=Single  exp_width=8  frac_width=24  explicit_period=off  period=1  equ=P=C  opselect=C  inp2=PCIN>>17  opr=+  inp1=P  carry=CIN  dbl_ovrd=off  block_type=constant
  fluff : xbsIndex_r4/Concat  num_inputs=2  dbl_ovrd=off  block_type=concat
  invert : xbsIndex_r4/Slice  nbits=1  boolean_output=on  mode=Upper Bit Location + Width  bit1=0  base1=MSB of Input  bit0=0  base0=LSB of Input  dbl_ovrd=off  block_type=slice
  lookup : xbsIndex_r4/Slice  nbits=3  boolean_output=off  mode=Lower Bit Location + Width  bit1=0  base1=MSB of Input  bit0=0  base0=LSB of Input  dbl_ovrd=off  block_type=slice
  new_add : xbsIndex_r4/Slice  nbits=4  boolean_output=off  mode=Lower Bit Location + Width  bit1=0  base1=MSB of Input  bit0=0  base0=LSB of Input  dbl_ovrd=off  block_type=slice
  pad : xbsIndex_r4/Constant  const=0  gui_display_data_type=Fixed-point  arith_type=Unsigned  n_bits=1  bin_pt=0  preci_type=Single  exp_width=8  frac_width=24  explicit_period=off  period=1  equ=P=C  opselect=C  inp2=PCIN>>17  opr=+  inp1=P  carry=CIN  dbl_ovrd=off  block_type=constant
  quadrant : xbsIndex_r4/Slice  nbits=2  boolean_output=off  mode=Upper Bit Location + Width  bit1=0  base1=MSB of Input  bit0=0  base0=LSB of Input  dbl_ovrd=off  block_type=slice
  negate : Outport
  add : Outport  Port=2
  misco : Outport  Port=3
  wires:
  theta/1 -> fluff/2
  pad/1 -> fluff/1
  fluff/1 -> quadrant/1, lookup/1
  direction_offset/1 -> AddSub5/1
  quadrant/1 -> AddSub5/2
  lookup/1 -> Concat/2
  AddSub5/1 -> Concat/1, invert/1
  Concat/1 -> new_add/1
  new_add/1 -> Delay14/1
  Convert2/1 -> add/1
  Delay14/1 -> Delay13/1
  Delay13/1 -> Convert2/1
  invert/1 -> Delay2/1
  Delay2/1 -> negate/1
  misci/1 -> Delay1/1
  Delay1/1 -> misco/1

== system rfsoc4x2_ospfb_128/fft2/fft_biplex/biplex_core/fft_stage_5/butterfly_direct/twiddle/coeff_gen/cosin/invert0 ==
  negate : Inport
  in : Inport  Port=2
  misci : Inport  Port=3
  Delay1 : xbsIndex_r4/Delay  rst=off  infoeditControl=Selection of Reset will increase slice count due to use of real FFs and instead of SRLs  en=off  latency=mux_latency+neg_latency  reg_retiming=on  dbl_ovrd=off  block_type=delay
  Delay20 : xbsIndex_r4/Delay  rst=off  infoeditControl=Selection of Reset will increase slice count due to use of real FFs and instead of SRLs  en=off  latency=neg_latency  reg_retiming=on  dbl_ovrd=off  block_type=delay
  Delay21 : xbsIndex_r4/Delay  rst=off  infoeditControl=Selection of Reset will increase slice count due to use of real FFs and instead of SRLs  en=off  latency=neg_latency  reg_retiming=on  dbl_ovrd=off  block_type=delay
  Negate : xbsIndex_r4/Negate  precision=User Defined  arith_type="Signed  (2's comp)"  n_bits=n_bits  bin_pt=bin_pt  quantization=Truncate  overflow=Saturate  en=off  latency=neg_latency  dbl_ovrd=off  block_type=negate
  mux : xbsIndex_r4/Mux  inputs=2  en=off  latency=mux_latency  precision=Full  arith_type=Unsigned  n_bits=16  bin_pt=14  quantization=Truncate  overflow=Wrap  dbl_ovrd=off  block_type=mux
  out : Outport
  misco : Outport  Port=2
  wires:
  misci/1 -> Delay1/1
  negate/1 -> Delay21/1
  in/1 -> Negate/1, Delay20/1
  Delay21/1 -> mux/1
  Delay20/1 -> mux/2
  Negate/1 -> mux/3
  mux/1 -> out/1
  Delay1/1 -> misco/1
